simulink model "second_lab"  (R2025b)
settings: Solver=VariableStepAuto  StartTime=0.0  StopTime=10.0  RelTol=1e-3
settings Model: Creator=reino  LastModifiedBy=reino

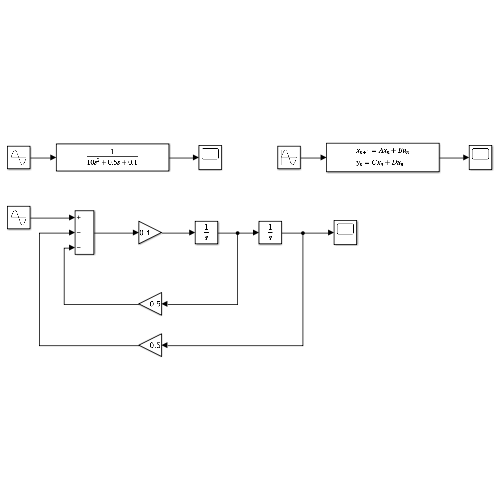
[thumbnail: Simulink's stored preview of the top-level diagram]
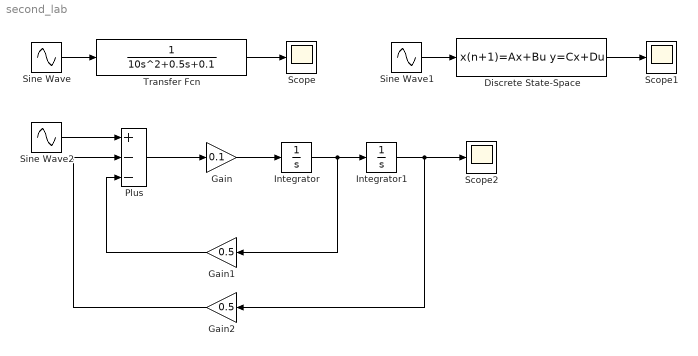
== system second_lab ==
  Discrete State-Space : DiscreteStateSpace  A=[0 1; -0.01 -0.05]  B=[0; 0.1]  C=[1 0]  D=0  SampleTime=-1
  Gain : Gain  Gain=0.1
  Gain1 : Gain  Gain=0.5
  Gain2 : Gain  Gain=0.5
  Integrator : Integrator
  Integrator1 : Integrator
  Plus : Sum  Inputs=+--
  Scope : Scope
  Scope1 : Scope
  Scope2 : Scope
      settings: DataLoggingVariableName=ScopeData2
  Sine Wave : Sin  SampleTime=0
  Sine Wave1 : Sin  SampleTime=0
  Sine Wave2 : Sin  SampleTime=0
  Transfer Fcn : TransferFcn  Denominator=[10 0.5 0.1]
  wires:
  Sine Wave/1 -> Transfer Fcn/1
  Transfer Fcn/1 -> Scope/1
  Sine Wave1/1 -> Discrete State-Space/1
  Discrete State-Space/1 -> Scope1/1
  Gain1/1 -> Plus/3
  Plus/1 -> Gain/1
  Gain/1 -> Integrator/1
  Integrator/1 -> Gain1/1, Integrator1/1
  Integrator1/1 -> Gain2/1, Scope2/1
  Sine Wave2/1 -> Plus/1
  Gain2/1 -> Plus/2
